simulink model "mars_rover_terrain"  (R2025a)
settings: Solver=daessc  StartTime=0.0  StopTime=130*10  FixedStep=1e-10  MaxStep=1e-1  RelTol=1e-3  AbsTol=1e-3  EnableMultiTasking=on
undefined symbols (not defined in the file): arm_q0, Control, eeConfig, L1, L2, L3, LS1, LS3, R1, R2, R3, Rover, rover_path, RS1, RS3, X, Y, Z
libraries: sm_lib x137, nesl_utility x109, fl_lib x85, sdl_lib x20, ee_lib x10, mars_rover_lib x8, simulink x4, slpidlib x3, batteryecm_lib x2, robotcorelib x1, robotalgslib x1
(part 3 of 10)

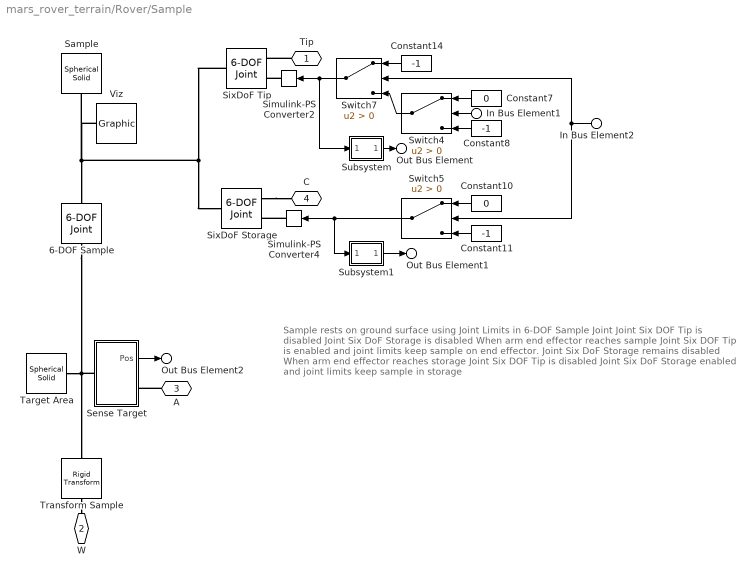
== system mars_rover_terrain/Rover/Sample ==
  note: Sample rests on ground surface using Joint Limits in 6-DOF Sample Joint
      | Joint Six DOF Tip is disabled
      | Joint Six DoF Storage is disabled
      |
      | When arm end effector reaches sample
      | Joint Six DOF Tip is enabled and joint limits keep sample on end effector.
      | Joint Six DoF Storage remains disabled
      |
      | When arm end effector reaches storage
      | Joint Six DOF Tip is disabled
      | Joint Six DoF Storage enabled and joint limits keep sample in storage
  In Bus Element1 : Inport  PortName=Ctrl  Element=Hold
  In Bus Element2 : Inport  PortName=Ctrl  Element=Stored
  6-DOF Sample : sm_lib/Joints/6-DOF Joint  JointMode=Normal  CompositeWrenchDir=FollowerOnBase  CompositeWrenchFrame=BaseFrame  SenseConstraintForce=off  SenseConstraintTorque=off  SenseTotalForce=off  SenseTotalTorque=off  PxPositionTargetSpecify=off  PxPositionTargetPriority=High  PxPositionTargetValue=0  PxPositionTargetValueUnits=m  PxVelocityTargetSpecify=off  PxVelocityTargetPriority=High  PxVelocityTargetValue=0  PxVelocityTargetValueUnits=m/s  PxEquilibriumPosition=0  PxEquilibriumPositionUnits=m  PxSpringStiffness=0  PxSpringStiffnessUnits=N/m  PxDampingCoefficient=0  PxDampingCoefficientUnits=N/(m/s)  PxLowerLimitSpecify=off  PxLowerLimitBound=-1  PxLowerLimitBoundUnits=m  PxLowerLimitStiffness=1e6  PxLowerLimitStiffnessUnits=N/m  PxLowerLimitDamping=1e3  PxLowerLimitDampingUnits=N/(m/s)  PxLowerLimitTransitionRegionWidth=1e-4  PxLowerLimitTransitionRegionWidthUnits=m  PxUpperLimitSpecify=off  PxUpperLimitBound=1  PxUpperLimitBoundUnits=m  PxUpperLimitStiffness=1e6  PxUpperLimitStiffnessUnits=N/m  PxUpperLimitDamping=1e3  PxUpperLimitDampingUnits=N/(m/s)  PxUpperLimitTransitionRegionWidth=1e-4  PxUpperLimitTransitionRegionWidthUnits=m  PxTorqueActuationMode=NoTorque  PxMotionActuationMode=ComputedMotion  PxSensePosition=off  PxSenseVelocity=off  PxSenseAcceleration=off  PxSenseTorqueForce=off  PxSenseLowerLimitTorqueForce=off  PxSenseUpperLimitTorqueForce=off  PyPositionTargetSpecify=off  PyPositionTargetPriority=High  PyPositionTargetValue=0  PyPositionTargetValueUnits=m  PyVelocityTargetSpecify=off  PyVelocityTargetPriority=High  PyVelocityTargetValue=0  PyVelocityTargetValueUnits=m/s  PyEquilibriumPosition=0  PyEquilibriumPositionUnits=m  PySpringStiffness=0  PySpringStiffnessUnits=N/m  PyDampingCoefficient=0  PyDampingCoefficientUnits=N/(m/s)  PyLowerLimitSpecify=off  PyLowerLimitBound=-1  PyLowerLimitBoundUnits=m  PyLowerLimitStiffness=1e6  PyLowerLimitStiffnessUnits=N/m  PyLowerLimitDamping=1e3  PyLowerLimitDampingUnits=N/(m/s)  PyLowerLimitTransitionRegionWidth=1e-4  PyLowerLimitTransitionRegionWidthUnits=m  PyUpperLimitSpecify=off  PyUpperLimitBound=1  PyUpperLimitBoundUnits=m  PyUpperLimitStiffness=1e6  PyUpperLimitStiffnessUnits=N/m  PyUpperLimitDamping=1e3  PyUpperLimitDampingUnits=N/(m/s)  PyUpperLimitTransitionRegionWidth=1e-4  PyUpperLimitTransitionRegionWidthUnits=m  PyTorqueActuationMode=NoTorque  PyMotionActuationMode=ComputedMotion  PySensePosition=off  PySenseVelocity=off  PySenseAcceleration=off  PySenseTorqueForce=off  PySenseLowerLimitTorqueForce=off  PySenseUpperLimitTorqueForce=off  PzPositionTargetSpecify=off  PzPositionTargetPriority=High  PzPositionTargetValue=0  PzPositionTargetValueUnits=m  PzVelocityTargetSpecify=off  PzVelocityTargetPriority=High  PzVelocityTargetValue=0  PzVelocityTargetValueUnits=m/s  PzEquilibriumPosition=0  PzEquilibriumPositionUnits=m  PzSpringStiffness=0  PzSpringStiffnessUnits=N/m  PzDampingCoefficient=0  PzDampingCoefficientUnits=N/(m/s)  PzLowerLimitSpecify=on  PzLowerLimitBound=0  PzLowerLimitBoundUnits=m  PzLowerLimitStiffness=1e6  PzLowerLimitStiffnessUnits=N/m  PzLowerLimitDamping=1e3  PzLowerLimitDampingUnits=N/(m/s)  PzLowerLimitTransitionRegionWidth=1e-4  PzLowerLimitTransitionRegionWidthUnits=m  PzUpperLimitSpecify=off  PzUpperLimitBound=1  PzUpperLimitBoundUnits=m  PzUpperLimitStiffness=1e6  PzUpperLimitStiffnessUnits=N/m  PzUpperLimitDamping=1e3  PzUpperLimitDampingUnits=N/(m/s)  PzUpperLimitTransitionRegionWidth=1e-4  PzUpperLimitTransitionRegionWidthUnits=m  PzTorqueActuationMode=NoTorque  PzMotionActuationMode=ComputedMotion  PzSensePosition=off  PzSenseVelocity=off  PzSenseAcceleration=off  PzSenseTorqueForce=off  PzSenseLowerLimitTorqueForce=off  PzSenseUpperLimitTorqueForce=off  SphPositionTargetSpecify=off  SphPositionTargetPriority=High  SphPositionTargetRotationMethod=None  SphPositionTargetFollAlignAxisA=+X  SphPositionTargetBaseAlignAxisA=+Y  SphPositionTargetFollAlignAxisB=+Y  SphPositionTargetBaseAlignAxisB=+Z  SphPositionTargetRotationStandardAxis=+Z  SphPositionTargetRotationAngle=0.0  SphPositionTargetRotationAngleUnits=deg  SphPositionTargetRotationArbitraryAxis=[0 0 1]  SphPositionTargetRotationSequenceAxes=FollowerAxes  SphPositionTargetRotationSequence=XYX  SphPositionTargetRotationSequenceAngles=[0 0 0]  SphPositionTargetRotationSequenceAnglesUnits=deg  SphPositionTargetRotationMatrix=[1 0 0; 0 1 0; 0 0 1]  SphPositionTargetQuaternion=[1 0 0 0]  SphVelocityTargetSpecify=off  SphVelocityTargetPriority=High  SphVelocityTargetValue=[0 0 0]  SphVelocityTargetValueUnits=deg/s  SphVelocityTargetInFollowerFrame=on  SphEqPosRotationMethod=None  SphEqPosFollAlignAxisA=+X  SphEqPosBaseAlignAxisA=+Y  SphEqPosFollAlignAxisB=+Y  SphEqPosBaseAlignAxisB=+Z  SphEqPosRotationStandardAxis=+Z  SphEqPosRotationAngle=0.0  SphEqPosRotationAngleUnits=deg  SphEqPosRotationArbitraryAxis=[0 0 1]  SphEqPosRotationSequenceAxes=FollowerAxes  SphEqPosRotationSequence=XYX  SphEqPosRotationSequenceAngles=[0 0 0]  SphEqPosRotationSequenceAnglesUnits=deg  SphEqPosRotationMatrix=[1 0 0; 0 1 0; 0 0 1]  SphEqPosQuaternion=[1 0 0 0]  SphSpringStiffness=0  SphSpringStiffnessUnits=N*m/deg  SphDampingCoefficient=0  SphDampingCoefficientUnits=N*m/(deg/s)  SphLowerLimitSpecify=off  SphLowerLimitBound=15  SphLowerLimitBoundUnits=deg  SphLowerLimitStiffness=1e4  SphLowerLimitStiffnessUnits=N*m/deg  SphLowerLimitDamping=10  SphLowerLimitDampingUnits=N*m/(deg/s)  SphLowerLimitTransitionRegionWidth=0.1  SphLowerLimitTransitionRegionWidthUnits=deg  SphUpperLimitSpecify=off  SphUpperLimitBound=45  SphUpperLimitBoundUnits=deg  SphUpperLimitStiffness=1e4  SphUpperLimitStiffnessUnits=N*m/deg  SphUpperLimitDamping=10  SphUpperLimitDampingUnits=N*m/(deg/s)  SphUpperLimitTransitionRegionWidth=0.1  SphUpperLimitTransitionRegionWidthUnits=deg  SphTorqueActuationMode=NoTorque  SphActuateTorqueX=off  SphActuateTorqueY=off  SphActuateTorqueZ=off  SphActuateTorque=off  SphActuationFrame=BaseFrame  SphSensePosition=off  SphSenseVelocityX=off  SphSenseVelocityY=off  SphSenseVelocityZ=off  SphSenseVelocity=off  SphSenseAccelerationX=off  SphSenseAccelerationY=off  SphSenseAccelerationZ=off  SphSenseAcceleration=off  SphSenseLowerLimitTorqueMag=off  SphSenseUpperLimitTorqueMag=off  SphSensingFrame=BaseFrame
  Constant10 : Constant  Value=0
  Constant11 : Constant  Value=-1
  Constant14 : Constant  Value=-1
  Constant7 : Constant  Value=0
  Constant8 : Constant  Value=-1
  Sample : sm_lib/Body Elements/Spherical Solid  SphereRadius=0.02  SphereRadiusUnits=m  ExportEntireGeometry=off  InertiaType=CalculateFromGeometry  BasedOnType=Density  Density=2582  DensityUnits=kg/m^3  Mass=0.001  MassUnits=kg  CenterOfMass=[0 0 0]  CenterOfMassUnits=m  MomentsOfInertia=[1 1 1]  MomentsOfInertiaUnits=kg*m^2  ProductsOfInertia=[0 0 0]  ProductsOfInertiaUnits=kg*m^2  GraphicType=FromGeometry  MarkerShape=Sphere  MarkerSize=10  GraphicVisPropType=AdvancedVisualProperties  GraphicDiffuseColor=[1 0 0]  GraphicOpacity=1.0  GraphicSpecularColor=[0.5 0.5 0.5 1.0]  GraphicAmbientColor=[0.15 0.15 0.15 1.0]  GraphicEmissiveColor=[0.0 0.0 0.0 1.0]  GraphicShininess=25  DoExposeReferenceFrame=on  SerializedFrames=<Frames/>
  Sense Target : Subsystem
  Simulink-PS Converter2 : nesl_utility/Simulink-PS Converter  PhysicalDomain=network_engine_domain  SubClassName=ps_input  LeftPortType=input  RightPortType=output  PseudoPeriodic=off  Frequencies=[]  NoiseDistribution=none  NoiseParameters=[]  Unit=1  AffineConversion=off  FilteringAndDerivatives=provide  SimscapeFilterOrder=1  InputFilterTimeConstant=0.001  UdotUserProvided=0
  Simulink-PS Converter4 : nesl_utility/Simulink-PS Converter  PhysicalDomain=network_engine_domain  SubClassName=ps_input  LeftPortType=input  RightPortType=output  PseudoPeriodic=off  Frequencies=[]  NoiseDistribution=none  NoiseParameters=[]  Unit=1  AffineConversion=off  FilteringAndDerivatives=provide  SimscapeFilterOrder=1  InputFilterTimeConstant=0.001  UdotUserProvided=0
  SixDoF Storage : sm_lib/Joints/6-DOF Joint  JointMode=ProvidedByInput  CompositeWrenchDir=FollowerOnBase  CompositeWrenchFrame=BaseFrame  SenseConstraintForce=off  SenseConstraintTorque=off  SenseTotalForce=off  SenseTotalTorque=off  PxPositionTargetSpecify=off  PxPositionTargetPriority=High  PxPositionTargetValue=0  PxPositionTargetValueUnits=m  PxVelocityTargetSpecify=off  PxVelocityTargetPriority=High  PxVelocityTargetValue=0  PxVelocityTargetValueUnits=m/s  PxEquilibriumPosition=0  PxEquilibriumPositionUnits=m  PxSpringStiffness=0  PxSpringStiffnessUnits=N/m  PxDampingCoefficient=0.1  PxDampingCoefficientUnits=N/(m/s)  PxLowerLimitSpecify=on  PxLowerLimitBound=-0.01  PxLowerLimitBoundUnits=m  PxLowerLimitStiffness=1e4  PxLowerLimitStiffnessUnits=N/m  PxLowerLimitDamping=1e2  PxLowerLimitDampingUnits=N/(m/s)  PxLowerLimitTransitionRegionWidth=1e-3  PxLowerLimitTransitionRegionWidthUnits=m  PxUpperLimitSpecify=on  PxUpperLimitBound=0.01  PxUpperLimitBoundUnits=m  PxUpperLimitStiffness=1e4  PxUpperLimitStiffnessUnits=N/m  PxUpperLimitDamping=1e2  PxUpperLimitDampingUnits=N/(m/s)  PxUpperLimitTransitionRegionWidth=1e-3  PxUpperLimitTransitionRegionWidthUnits=m  PxTorqueActuationMode=NoTorque  PxMotionActuationMode=ComputedMotion  PxSensePosition=off  PxSenseVelocity=off  PxSenseAcceleration=off  PxSenseTorqueForce=off  PxSenseLowerLimitTorqueForce=off  PxSenseUpperLimitTorqueForce=off  PyPositionTargetSpecify=off  PyPositionTargetPriority=High  PyPositionTargetValue=0  PyPositionTargetValueUnits=m  PyVelocityTargetSpecify=off  PyVelocityTargetPriority=High  PyVelocityTargetValue=0  PyVelocityTargetValueUnits=m/s  PyEquilibriumPosition=0  PyEquilibriumPositionUnits=m  PySpringStiffness=0  PySpringStiffnessUnits=N/m  PyDampingCoefficient=0.1  PyDampingCoefficientUnits=N/(m/s)  PyLowerLimitSpecify=on  PyLowerLimitBound=-0.01  PyLowerLimitBoundUnits=m  PyLowerLimitStiffness=1e4  PyLowerLimitStiffnessUnits=N/m  PyLowerLimitDamping=1e3  PyLowerLimitDampingUnits=N/(m/s)  PyLowerLimitTransitionRegionWidth=1e-3  PyLowerLimitTransitionRegionWidthUnits=m  PyUpperLimitSpecify=on  PyUpperLimitBound=0.01  PyUpperLimitBoundUnits=m  PyUpperLimitStiffness=1e4  PyUpperLimitStiffnessUnits=N/m  PyUpperLimitDamping=1e3  PyUpperLimitDampingUnits=N/(m/s)  PyUpperLimitTransitionRegionWidth=1e-3  PyUpperLimitTransitionRegionWidthUnits=m  PyTorqueActuationMode=NoTorque  PyMotionActuationMode=ComputedMotion  PySensePosition=off  PySenseVelocity=off  PySenseAcceleration=off  PySenseTorqueForce=off  PySenseLowerLimitTorqueForce=off  PySenseUpperLimitTorqueForce=off  PzPositionTargetSpecify=off  PzPositionTargetPriority=High  PzPositionTargetValue=0  PzPositionTargetValueUnits=m  PzVelocityTargetSpecify=off  PzVelocityTargetPriority=High  PzVelocityTargetValue=0  PzVelocityTargetValueUnits=m/s  PzEquilibriumPosition=0  PzEquilibriumPositionUnits=m  PzSpringStiffness=0  PzSpringStiffnessUnits=N/m  PzDampingCoefficient=0.1  PzDampingCoefficientUnits=N/(m/s)  PzLowerLimitSpecify=on  PzLowerLimitBound=-0.02  PzLowerLimitBoundUnits=m  PzLowerLimitStiffness=1e4  PzLowerLimitStiffnessUnits=N/m  PzLowerLimitDamping=1e3  PzLowerLimitDampingUnits=N/(m/s)  PzLowerLimitTransitionRegionWidth=1e-3  PzLowerLimitTransitionRegionWidthUnits=m  PzUpperLimitSpecify=on  PzUpperLimitBound=0.02  PzUpperLimitBoundUnits=m  PzUpperLimitStiffness=1e4  PzUpperLimitStiffnessUnits=N/m  PzUpperLimitDamping=1e3  PzUpperLimitDampingUnits=N/(m/s)  PzUpperLimitTransitionRegionWidth=1e-3  PzUpperLimitTransitionRegionWidthUnits=m  PzTorqueActuationMode=NoTorque  PzMotionActuationMode=ComputedMotion  PzSensePosition=off  PzSenseVelocity=off  PzSenseAcceleration=off  PzSenseTorqueForce=off  PzSenseLowerLimitTorqueForce=off  PzSenseUpperLimitTorqueForce=off  SphPositionTargetSpecify=off  SphPositionTargetPriority=High  SphPositionTargetRotationMethod=None  SphPositionTargetFollAlignAxisA=+X  SphPositionTargetBaseAlignAxisA=+Y  SphPositionTargetFollAlignAxisB=+Y  SphPositionTargetBaseAlignAxisB=+Z  SphPositionTargetRotationStandardAxis=+Z  SphPositionTargetRotationAngle=0.0  SphPositionTargetRotationAngleUnits=deg  SphPositionTargetRotationArbitraryAxis=[0 0 1]  SphPositionTargetRotationSequenceAxes=FollowerAxes  SphPositionTargetRotationSequence=XYX  SphPositionTargetRotationSequenceAngles=[0 0 0]  SphPositionTargetRotationSequenceAnglesUnits=deg  SphPositionTargetRotationMatrix=[1 0 0; 0 1 0; 0 0 1]  SphPositionTargetQuaternion=[1 0 0 0]  SphVelocityTargetSpecify=off  SphVelocityTargetPriority=High  SphVelocityTargetValue=[0 0 0]  SphVelocityTargetValueUnits=deg/s  SphVelocityTargetInFollowerFrame=on  SphEqPosRotationMethod=None  SphEqPosFollAlignAxisA=+X  SphEqPosBaseAlignAxisA=+Y  SphEqPosFollAlignAxisB=+Y  SphEqPosBaseAlignAxisB=+Z  SphEqPosRotationStandardAxis=+Z  SphEqPosRotationAngle=0.0  SphEqPosRotationAngleUnits=deg  SphEqPosRotationArbitraryAxis=[0 0 1]  SphEqPosRotationSequenceAxes=FollowerAxes  SphEqPosRotationSequence=XYX  SphEqPosRotationSequenceAngles=[0 0 0]  SphEqPosRotationSequenceAnglesUnits=deg  SphEqPosRotationMatrix=[1 0 0; 0 1 0; 0 0 1]  SphEqPosQuaternion=[1 0 0 0]  SphSpringStiffness=0  SphSpringStiffnessUnits=N*m/deg  SphDampingCoefficient=0.1  SphDampingCoefficientUnits=N*m/(deg/s)  SphLowerLimitSpecify=off  SphLowerLimitBound=15  SphLowerLimitBoundUnits=deg  SphLowerLimitStiffness=1e4  SphLowerLimitStiffnessUnits=N*m/deg  SphLowerLimitDamping=10  SphLowerLimitDampingUnits=N*m/(deg/s)  SphLowerLimitTransitionRegionWidth=0.1  SphLowerLimitTransitionRegionWidthUnits=deg  SphUpperLimitSpecify=off  SphUpperLimitBound=45  SphUpperLimitBoundUnits=deg  SphUpperLimitStiffness=1e4  SphUpperLimitStiffnessUnits=N*m/deg  SphUpperLimitDamping=10  SphUpperLimitDampingUnits=N*m/(deg/s)  SphUpperLimitTransitionRegionWidth=0.1  SphUpperLimitTransitionRegionWidthUnits=deg  SphTorqueActuationMode=NoTorque  SphActuateTorqueX=off  SphActuateTorqueY=off  SphActuateTorqueZ=off  SphActuateTorque=off  SphActuationFrame=BaseFrame  SphSensePosition=off  SphSenseVelocityX=off  SphSenseVelocityY=off  SphSenseVelocityZ=off  SphSenseVelocity=off  SphSenseAccelerationX=off  SphSenseAccelerationY=off  SphSenseAccelerationZ=off  SphSenseAcceleration=off  SphSenseLowerLimitTorqueMag=off  SphSenseUpperLimitTorqueMag=off  SphSensingFrame=BaseFrame
  SixDoF Tip : sm_lib/Joints/6-DOF Joint  JointMode=ProvidedByInput  CompositeWrenchDir=FollowerOnBase  CompositeWrenchFrame=BaseFrame  SenseConstraintForce=off  SenseConstraintTorque=off  SenseTotalForce=off  SenseTotalTorque=off  PxPositionTargetSpecify=off  PxPositionTargetPriority=High  PxPositionTargetValue=0  PxPositionTargetValueUnits=m  PxVelocityTargetSpecify=off  PxVelocityTargetPriority=High  PxVelocityTargetValue=0  PxVelocityTargetValueUnits=m/s  PxEquilibriumPosition=0  PxEquilibriumPositionUnits=m  PxSpringStiffness=0  PxSpringStiffnessUnits=N/m  PxDampingCoefficient=0.1  PxDampingCoefficientUnits=N/(m/s)  PxLowerLimitSpecify=on  PxLowerLimitBound=-Rover.Arm.Tip.lim.bound  PxLowerLimitBoundUnits=m  PxLowerLimitStiffness=Rover.Arm.Tip.lim.k  PxLowerLimitStiffnessUnits=N/m  PxLowerLimitDamping=Rover.Arm.Tip.lim.d  PxLowerLimitDampingUnits=N/(m/s)  PxLowerLimitTransitionRegionWidth=Rover.Arm.Tip.lim.w  PxLowerLimitTransitionRegionWidthUnits=m  PxUpperLimitSpecify=on  PxUpperLimitBound=Rover.Arm.Tip.lim.bound  PxUpperLimitBoundUnits=m  PxUpperLimitStiffness=Rover.Arm.Tip.lim.k  PxUpperLimitStiffnessUnits=N/m  PxUpperLimitDamping=Rover.Arm.Tip.lim.d  PxUpperLimitDampingUnits=N/(m/s)  PxUpperLimitTransitionRegionWidth=Rover.Arm.Tip.lim.w  PxUpperLimitTransitionRegionWidthUnits=m  PxTorqueActuationMode=NoTorque  PxMotionActuationMode=ComputedMotion  PxSensePosition=off  PxSenseVelocity=off  PxSenseAcceleration=off  PxSenseTorqueForce=off  PxSenseLowerLimitTorqueForce=off  PxSenseUpperLimitTorqueForce=off  PyPositionTargetSpecify=off  PyPositionTargetPriority=High  PyPositionTargetValue=0  PyPositionTargetValueUnits=m  PyVelocityTargetSpecify=off  PyVelocityTargetPriority=High  PyVelocityTargetValue=0  PyVelocityTargetValueUnits=m/s  PyEquilibriumPosition=0  PyEquilibriumPositionUnits=m  PySpringStiffness=0  PySpringStiffnessUnits=N/m  PyDampingCoefficient=0.1  PyDampingCoefficientUnits=N/(m/s)  PyLowerLimitSpecify=on  PyLowerLimitBound=-Rover.Arm.Tip.lim.bound  PyLowerLimitBoundUnits=m  PyLowerLimitStiffness=Rover.Arm.Tip.lim.k  PyLowerLimitStiffnessUnits=N/m  PyLowerLimitDamping=Rover.Arm.Tip.lim.d  PyLowerLimitDampingUnits=N/(m/s)  PyLowerLimitTransitionRegionWidth=Rover.Arm.Tip.lim.w  PyLowerLimitTransitionRegionWidthUnits=m  PyUpperLimitSpecify=on  PyUpperLimitBound=Rover.Arm.Tip.lim.bound  PyUpperLimitBoundUnits=m  PyUpperLimitStiffness=Rover.Arm.Tip.lim.k  PyUpperLimitStiffnessUnits=N/m  PyUpperLimitDamping=Rover.Arm.Tip.lim.d  PyUpperLimitDampingUnits=N/(m/s)  PyUpperLimitTransitionRegionWidth=Rover.Arm.Tip.lim.w  PyUpperLimitTransitionRegionWidthUnits=m  PyTorqueActuationMode=NoTorque  PyMotionActuationMode=ComputedMotion  PySensePosition=off  PySenseVelocity=off  PySenseAcceleration=off  PySenseTorqueForce=off  PySenseLowerLimitTorqueForce=off  PySenseUpperLimitTorqueForce=off  PzPositionTargetSpecify=off  PzPositionTargetPriority=High  PzPositionTargetValue=0  PzPositionTargetValueUnits=m  PzVelocityTargetSpecify=off  PzVelocityTargetPriority=High  PzVelocityTargetValue=0  PzVelocityTargetValueUnits=m/s  PzEquilibriumPosition=0  PzEquilibriumPositionUnits=m  PzSpringStiffness=0  PzSpringStiffnessUnits=N/m  PzDampingCoefficient=0.1  PzDampingCoefficientUnits=N/(m/s)  PzLowerLimitSpecify=on  PzLowerLimitBound=-Rover.Arm.Tip.lim.bound  PzLowerLimitBoundUnits=m  PzLowerLimitStiffness=Rover.Arm.Tip.lim.k  PzLowerLimitStiffnessUnits=N/m  PzLowerLimitDamping=Rover.Arm.Tip.lim.d  PzLowerLimitDampingUnits=N/(m/s)  PzLowerLimitTransitionRegionWidth=Rover.Arm.Tip.lim.w  PzLowerLimitTransitionRegionWidthUnits=m  PzUpperLimitSpecify=on  PzUpperLimitBound=Rover.Arm.Tip.lim.bound  PzUpperLimitBoundUnits=m  PzUpperLimitStiffness=Rover.Arm.Tip.lim.k  PzUpperLimitStiffnessUnits=N/m  PzUpperLimitDamping=Rover.Arm.Tip.lim.d  PzUpperLimitDampingUnits=N/(m/s)  PzUpperLimitTransitionRegionWidth=Rover.Arm.Tip.lim.w  PzUpperLimitTransitionRegionWidthUnits=m  PzTorqueActuationMode=NoTorque  PzMotionActuationMode=ComputedMotion  PzSensePosition=off  PzSenseVelocity=off  PzSenseAcceleration=off  PzSenseTorqueForce=off  PzSenseLowerLimitTorqueForce=off  PzSenseUpperLimitTorqueForce=off  SphPositionTargetSpecify=off  SphPositionTargetPriority=High  SphPositionTargetRotationMethod=None  SphPositionTargetFollAlignAxisA=+X  SphPositionTargetBaseAlignAxisA=+Y  SphPositionTargetFollAlignAxisB=+Y  SphPositionTargetBaseAlignAxisB=+Z  SphPositionTargetRotationStandardAxis=+Z  SphPositionTargetRotationAngle=0.0  SphPositionTargetRotationAngleUnits=deg  SphPositionTargetRotationArbitraryAxis=[0 0 1]  SphPositionTargetRotationSequenceAxes=FollowerAxes  SphPositionTargetRotationSequence=XYX  SphPositionTargetRotationSequenceAngles=[0 0 0]  SphPositionTargetRotationSequenceAnglesUnits=deg  SphPositionTargetRotationMatrix=[1 0 0; 0 1 0; 0 0 1]  SphPositionTargetQuaternion=[1 0 0 0]  SphVelocityTargetSpecify=off  SphVelocityTargetPriority=High  SphVelocityTargetValue=[0 0 0]  SphVelocityTargetValueUnits=deg/s  SphVelocityTargetInFollowerFrame=on  SphEqPosRotationMethod=None  SphEqPosFollAlignAxisA=+X  SphEqPosBaseAlignAxisA=+Y  SphEqPosFollAlignAxisB=+Y  SphEqPosBaseAlignAxisB=+Z  SphEqPosRotationStandardAxis=+Z  SphEqPosRotationAngle=0.0  SphEqPosRotationAngleUnits=deg  SphEqPosRotationArbitraryAxis=[0 0 1]  SphEqPosRotationSequenceAxes=FollowerAxes  SphEqPosRotationSequence=XYX  SphEqPosRotationSequenceAngles=[0 0 0]  SphEqPosRotationSequenceAnglesUnits=deg  SphEqPosRotationMatrix=[1 0 0; 0 1 0; 0 0 1]  SphEqPosQuaternion=[1 0 0 0]  SphSpringStiffness=0  SphSpringStiffnessUnits=N*m/deg  SphDampingCoefficient=0  SphDampingCoefficientUnits=N*m/(deg/s)  SphLowerLimitSpecify=off  SphLowerLimitBound=15  SphLowerLimitBoundUnits=deg  SphLowerLimitStiffness=1e4  SphLowerLimitStiffnessUnits=N*m/deg  SphLowerLimitDamping=10  SphLowerLimitDampingUnits=N*m/(deg/s)  SphLowerLimitTransitionRegionWidth=0.1  SphLowerLimitTransitionRegionWidthUnits=deg  SphUpperLimitSpecify=off  SphUpperLimitBound=45  SphUpperLimitBoundUnits=deg  SphUpperLimitStiffness=1e4  SphUpperLimitStiffnessUnits=N*m/deg  SphUpperLimitDamping=10  SphUpperLimitDampingUnits=N*m/(deg/s)  SphUpperLimitTransitionRegionWidth=0.1  SphUpperLimitTransitionRegionWidthUnits=deg  SphTorqueActuationMode=NoTorque  SphActuateTorqueX=off  SphActuateTorqueY=off  SphActuateTorqueZ=off  SphActuateTorque=off  SphActuationFrame=BaseFrame  SphSensePosition=off  SphSenseVelocityX=off  SphSenseVelocityY=off  SphSenseVelocityZ=off  SphSenseVelocity=off  SphSenseAccelerationX=off  SphSenseAccelerationY=off  SphSenseAccelerationZ=off  SphSenseAcceleration=off  SphSenseLowerLimitTorqueMag=off  SphSenseUpperLimitTorqueMag=off  SphSensingFrame=BaseFrame
  Subsystem : Subsystem
  Subsystem1 : Subsystem
  Switch4 : Switch  Criteria=u2 > Threshold  SaturateOnIntegerOverflow=off  InputSameDT=off
  Switch5 : Switch  Criteria=u2 > Threshold  SaturateOnIntegerOverflow=off  InputSameDT=off
  Switch7 : Switch  Criteria=u2 > Threshold  SaturateOnIntegerOverflow=off  InputSameDT=off
  Target Area : sm_lib/Body Elements/Spherical Solid  SphereRadius=0.35  SphereRadiusUnits=m  ExportEntireGeometry=off  InertiaType=CalculateFromGeometry  BasedOnType=Density  Density=1000  DensityUnits=kg/m^3  Mass=1  MassUnits=kg  CenterOfMass=[0 0 0]  CenterOfMassUnits=m  MomentsOfInertia=[1 1 1]  MomentsOfInertiaUnits=kg*m^2  ProductsOfInertia=[0 0 0]  ProductsOfInertiaUnits=kg*m^2  GraphicType=FromGeometry  MarkerShape=Sphere  MarkerSize=10  GraphicVisPropType=SimpleVisualProperties  GraphicDiffuseColor=[0.4 1.0 0.2]  GraphicOpacity=0.3  GraphicSpecularColor=[0.5 0.5 0.5 1.0]  GraphicAmbientColor=[0.15 0.15 0.15 1.0]  GraphicEmissiveColor=[0.0 0.0 0.0 1.0]  GraphicShininess=75  DoExposeReferenceFrame=on  SerializedFrames=<Frames/>
  Transform Sample : sm_lib/Frames and Transforms/Rigid Transform  RotationMethod=None  FollAlignAxisA=+X  BaseAlignAxisA=+Y  FollAlignAxisB=+Y  BaseAlignAxisB=+Z  RotationStandardAxis=+Z  RotationAngle=0.0  RotationAngleUnits=deg  RotationArbitraryAxis=[0 0 1]  RotationSequenceAxes=FollowerAxes  RotationSequence=XYX  RotationSequenceAngles=[0 0 0]  RotationSequenceAnglesUnits=deg  RotationMatrix=[1 0 0; 0 1 0; 0 0 1]  Quaternion=[1 0 0 0]  TranslationMethod=Cartesian  TranslationCartesianOffset=sample_position  TranslationCartesianOffsetUnits=m  TranslationStandardAxis=+Z  TranslationStandardOffset=0  TranslationStandardOffsetUnits=m  TranslationROffset=0  TranslationROffsetUnits=m  TranslationThetaOffset=0  TranslationThetaOffsetUnits=deg  TranslationZOffset=0  TranslationZOffsetUnits=m
  Viz : sm_lib/Body Elements/Graphic  GraphicType=Marker  MarkerShape=Frame  MarkerSize=5  GraphicVisPropType=SimpleVisualProperties  GraphicDiffuseColor=[1 0 0]  GraphicOpacity=1.0  GraphicSpecularColor=[0.5 0.5 0.5 1.0]  GraphicAmbientColor=[0.15 0.15 0.15 1.0]  GraphicEmissiveColor=[0.0 0.0 0.0 1.0]  GraphicShininess=75
  Tip : PMIOPort  Side=Right
  W : PMIOPort  Port=2  Side=Left
  A : PMIOPort  Port=3  Side=Right
  C : PMIOPort  Port=4  Side=Right
  Out Bus Element : Outport  PortName=m  Element=SampleTip
  Out Bus Element1 : Outport  PortName=m  Element=SampleStorage
  Out Bus Element2 : Outport  PortName=m  Element=TargetChassis
  wires:
  Constant7/1 -> Switch4/1
  Constant8/1 -> Switch4/3
  In Bus Element2/1 -> Switch5/2, Switch7/2
  Constant11/1 -> Switch5/3
  Constant10/1 -> Switch5/1
  Switch4/1 -> Switch7/3
  Switch5/1 -> Subsystem1/1(In1), Simulink-PS Converter4/1
  In Bus Element1/1 -> Switch4/2
  Constant14/1 -> Switch7/1
  Switch7/1 -> Subsystem/1(In1), Simulink-PS Converter2/1
  Subsystem/1(Out1) -> Out Bus Element/1
  Sense Target/1(Pos) -> Out Bus Element2/1
  Subsystem1/1(m) -> Out Bus Element1/1
  connections:
  SixDoF Tip/RConn1 -- Viz/RConn1 -- Sample/RConn1 -- 6-DOF Sample/RConn1 -- SixDoF Storage/RConn1
  Simulink-PS Converter4/RConn1 -- SixDoF Storage/LConn2
  SixDoF Storage/LConn1 -- C/RConn1
  6-DOF Sample/LConn1 -- Target Area/RConn1 -- Transform Sample/RConn1 -- Sense Target/LConn1
  Simulink-PS Converter2/RConn1 -- SixDoF Tip/LConn2
  Tip/RConn1 -- SixDoF Tip/LConn1
  A/RConn1 -- Sense Target/RConn1
  Transform Sample/LConn1 -- W/RConn1

== system mars_rover_terrain/Rover/Terrain ==
  note: Uncomment for additional terrain visualization options.
  Contact : Subsystem  mask{contact_k=Rover.Wheel_Surface.Contact.k, contact_d=Rover.Wheel_Surface.Contact.d, contact_tw=Rover.Wheel_Surface.Contact.trans_depth, friction_mus=Rover.Wheel_Surface.Friction.mu_static, friction_mud=Rover.Wheel_Surface.Friction.mu_dynamic, friction_vcrit=Rover.Wheel_Surface.Friction.vel_crit}
      mask prompts: contact_k "Stiffness (N/m)"; contact_d "Damping (N/(m/s))"; contact_tw "Transition Region Width (m)"; friction_mus "Coefficient of Static Friction"; friction_mud "Coefficient of Dynamic Friction"; friction_vcrit "Critical Velocity (m/s)"
      mask DialogControl cont_contact Prompt: Contact Parameters
      mask DialogControl cont_friction Prompt: Contact Friction
  Terrain Geometry : sm_lib/Body Elements/File Solid  Commented=on  ExtGeomFileName=mars_terrain.stl  UnitType=Custom  ExtGeomFileUnits=m  StepReaderType=HEX  ExportConvexHullGeometry=off  InertiaType=CalculateFromGeometry  BasedOnType=Mass  Density=1000  DensityUnits=kg/m^3  Mass=1  MassUnits=kg  CenterOfMass=[0 0 0]  CenterOfMassUnits=m  MomentsOfInertia=[1 1 1]  MomentsOfInertiaUnits=kg*m^2  ProductsOfInertia=[0 0 0]  ProductsOfInertiaUnits=kg*m^2  GraphicType=FromGeometry  MarkerShape=Sphere  MarkerSize=10  GraphicVisPropType=SimpleVisualProperties  GraphicDiffuseColor=[1.0 0.6 0.6]  GraphicOpacity=1.0  GraphicSpecularColor=[0.5 0.5 0.5 1.0]  GraphicAmbientColor=[0.15 0.15 0.15 1.0]  GraphicEmissiveColor=[0.0 0.0 0.0 1.0]  GraphicShininess=75  DoExposeReferenceFrame=on  SerializedFrames=<Frames/>
  Terrain Point Cloud : sm_lib/Curves and Surfaces/Point Cloud  Commented=on  CoordinatesMatrix=mars_terrain_grid.ptcloud  CoordinatesMatrixUnits=m  GraphicType=MarkerCloud  GraphicSphereRadius=0.03  GraphicSphereRadiusUnits=m  GraphicVisPropType=SimpleVisualProperties  GraphicDiffuseColor=[0 1 0]  GraphicOpacity=1.0  GraphicSpecularColor=[0.5 0.5 0.5 1.0]  GraphicAmbientColor=[0.15 0.15 0.15 1.0]  GraphicEmissiveColor=[0.0 0.0 0.0 1.0]  GraphicShininess=75
  Terrain Grid Surface : sm_lib/Curves and Surfaces/Grid Surface  XGridVector=mars_terrain_grid.xg  XGridVectorUnits=m  YGridVector=mars_terrain_grid.yg  YGridVectorUnits=m  ZHeights=mars_terrain_grid.z_heights  ZHeightsUnits=m  GraphicType=FromGeometry  GraphicVisPropType=SimpleVisualProperties  GraphicDiffuseColor=[187 109 63]/255*1.3  GraphicOpacity=1  GraphicSpecularColor=[0.5 0.5 0.5 1.0]  GraphicAmbientColor=[0.15 0.15 0.15 1.0]  GraphicEmissiveColor=[0.0 0.0 0.0 1.0]  GraphicShininess=75
  W : PMIOPort  Side=Right
  G : PMIOPort  Port=2  Side=Right
  connections:
  W/RConn1 -- Terrain Point Cloud/LConn1 -- Terrain Geometry/RConn1 -- Terrain Grid Surface/LConn1
  Contact/RConn1 -- G/RConn1
  Contact/RConn2 -- Terrain Grid Surface/RConn1

== system mars_rover_terrain/Control/Arm Control/ Trajectory Planner ==
  RoverAtGoal : Inport
  In Bus Element1 : Inport  Port=2  PortName=Sensing  Element=SampleTip
  In Bus Element2 : Inport  Port=2  PortName=Sensing  Element=SampleStorage
  In Bus Element3 : Inport  Port=2  PortName=Sensing  Element=TargetChassis
  Arm Angles : Inport  Port=3
  Check Drift : Subsystem
  Delay Arm Movement : Delay
  Delay Sample Check : Delay
  Planner Subsystem : Subsystem
  SampleDropOffCmdLogic : Subsystem
  SampleLoc wrt arm base : Subsystem
  SamplePickUpCmdLogic : Subsystem
  Scope : Scope  NumInputPorts=2
      settings: ActiveDisplayYMinimum=-0.125  ActiveDisplayYMaximum=1.125
  Switch : Switch  Criteria=u2 > Threshold  SaturateOnIntegerOverflow=off  InputSameDT=off
  hold1 : Subsystem
  hold2 : Subsystem
  q0 Arm : Constant  Value=arm_q0
  Hold : Outport
  Stored : Outport  Port=2
  Location : Outport  Port=3
  Mode : Outport  Port=4
  Cmd Angles : Outport  Port=5
  wires:
  Switch/1 -> Cmd Angles/1
  q0 Arm/1 -> Switch/3
  In Bus Element3/1 -> SampleLoc wrt arm base/2(SampleLoc), Check Drift/1(Sensor)
  Delay Arm Movement/1 -> Switch/2
  Arm Angles/1 -> Planner Subsystem/1(qJoints)
  SampleLoc wrt arm base/1(SamplePos) -> Check Drift/2(IK Target), Location/1, Planner Subsystem/2(SamplePosition)
  Planner Subsystem/2(CmdHold) -> SamplePickUpCmdLogic/1(u)
  Planner Subsystem/3(CmdStored) -> SampleDropOffCmdLogic/1(u)
  In Bus Element1/1 -> hold2/1(Enable)
  In Bus Element2/1 -> hold1/1(Enable)
  Planner Subsystem/1(qCmd) -> Switch/1
  hold2/1(plan) -> Planner Subsystem/3(Hold)
  hold1/1(plan) -> Planner Subsystem/4(Stored)
  SampleDropOffCmdLogic/1(y) -> Scope/2, Stored/1
  SamplePickUpCmdLogic/1(y) -> Scope/1, Hold/1
  Delay Sample Check/1 -> SampleLoc wrt arm base/1(Enable), Delay Arm Movement/1, Planner Subsystem/Enable
  RoverAtGoal/1 -> Delay Sample Check/1
  Planner Subsystem/4(Rover Mode) -> Mode/1

== system mars_rover_terrain/Control/Arm Control/Bus to Vec q ==
  B : Inport
  Bus Selector : BusSelector  OutputSignals=q.q1,q.q2,q.q3,q.q4,q.q5,q.q6
  Mux : Mux  Inputs=6
  V : Outport
  wires:
  Bus Selector/6 -> Mux/6  "<q6>"
  Bus Selector/4 -> Mux/4  "<q4>"
  Mux/1 -> V/1
  B/1 -> Bus Selector/1
  Bus Selector/1 -> Mux/1  "<q1>"
  Bus Selector/3 -> Mux/3  "<q3>"
  Bus Selector/2 -> Mux/2  "<q2>"
  Bus Selector/5 -> Mux/5  "<q5>"

== system mars_rover_terrain/Control/Arm Control/Vec to Bus q ==
  V : Inport
  Bus Creator : BusCreator  Inputs=6
  Demux : Demux  Outputs=6
  B : Outport
  wires:
  Demux/3 -> Bus Creator/3  "q3"
  Bus Creator/1 -> B/1
  V/1 -> Demux/1
  Demux/4 -> Bus Creator/4  "q4"
  Demux/1 -> Bus Creator/1  "q1"
  Demux/6 -> Bus Creator/6  "q6"
  Demux/2 -> Bus Creator/2  "q2"
  Demux/5 -> Bus Creator/5  "q5"

== system mars_rover_terrain/Control/Arm Control/Vec to Bus trq ==
  V : Inport
  Bus Creator : BusCreator  Inputs=6
  Demux : Demux  Outputs=6
  B : Outport
  wires:
  Demux/5 -> Bus Creator/5  "t5"
  Demux/2 -> Bus Creator/2  "t2"
  Demux/6 -> Bus Creator/6  "t6"
  Demux/1 -> Bus Creator/1  "t1"
  Demux/4 -> Bus Creator/4  "t4"
  V/1 -> Demux/1
  Bus Creator/1 -> B/1
  Demux/3 -> Bus Creator/3  "t3"

== system mars_rover_terrain/Control/Chassis Control/Ackerman Steer Angle ==
  note: ROC: Radius of Curvature
      | A3: Axle 3
      | L3: Rear Left Wheel
      | R3: Rear Right Wheel
  AtGoal : Inport
  Delta : Inport  Port=2
  Ackerman Steering Angle Formulation : MATLAB Function  TreatAsAtomicUnit=on
  Clock1 : Clock
  Constant : Constant  Value=Rover.Chassis.Length/2
  Constant3 : Constant  Value=0
  Constant4 : Constant  Value=Rover.Chassis.Width
  Gain3 : Gain  Gain=-1
  Gain4 : Gain  Gain=-1
  Hold Steer at Goal : Subsystem  TreatAsAtomicUnit=on
  Mux : Mux
  NOT : Logic  Operator=NOT  IconShape=distinctive  AllPortsSameDT=off  OutDataTypeStr=boolean
  Saturation{1..4} (4 alike) : Saturate  UpperLimit=60  LowerLimit=-60
  Scope : Scope  NumInputPorts=3
      settings: ActiveDisplayYMinimum=-35.60933  ActiveDisplayYMaximum=51.25577  DataLoggingVariableName=ScopeData2
  Switch2 : Switch  Criteria=u2 > Threshold  Threshold=1  SaturateOnIntegerOverflow=off  InputSameDT=off
  AckSteerAngs : Outport
  A3 ROC : Outport  Port=2
  L3ROC : Outport  Port=3
  R3ROC : Outport  Port=4
  wires:
  Delta/1 -> Switch2/1
  Ackerman Steering Angle Formulation/2(qSteerR3) -> Scope/3, Saturation3/1, Gain4/1
  Ackerman Steering Angle Formulation/5(R_R) -> R3ROC/1
  Saturation4/1 -> Mux/4  "R1"
  Saturation1/1 -> Mux/2  "L1"
  Hold Steer at Goal/1(d_h) -> Scope/1, Ackerman Steering Angle Formulation/1(delta)
  Ackerman Steering Angle Formulation/1(qSteerL3) -> Scope/2, Saturation2/1, Gain3/1
  Constant/1 -> Ackerman Steering Angle Formulation/2(L)
  Saturation3/1 -> Mux/3  "R3"
  Mux/1 -> AckSteerAngs/1
  Clock1/1 -> Switch2/2
  Switch2/1 -> Hold Steer at Goal/1(d)
  Gain4/1 -> Saturation4/1
  Saturation2/1 -> Mux/1  "L3"
  Constant4/1 -> Ackerman Steering Angle Formulation/3(d)
  Gain3/1 -> Saturation1/1
  Ackerman Steering Angle Formulation/4(L_R) -> L3ROC/1
  Ackerman Steering Angle Formulation/3(R) -> A3 ROC/1
  Constant3/1 -> Switch2/3
  AtGoal/1 -> NOT/1
  NOT/1 -> Hold Steer at Goal/Enable

== system mars_rover_terrain/Control/Chassis Control/Steering Controller ==
  Meas : Inport
  qSteerWhl : Inport  Port=2
  RoverAtGoal : Inport  Port=3
  Add : Sum  Inputs=+-
  Bus to Vec : Subsystem
  Check Difference : Subsystem
  Constant : Constant  Value=[Kp Ki]
  Constant1 : Constant  Value=[10 1 ]
  Constant2 : Constant  Value=Kd
  Constant3 : Constant  Value=N
  Demux : Demux  Outputs=2
  Demux1 : Demux
  Filter qMeas : Subsystem  mask(First-order lag supporting vector signals){b=[1 1 1 1]*Ts_Measq, x_initial=[0 0 0 0]}
      mask prompts: b "Filter time constant"; x_initial "Initial output"
      mask help: Models a lag of the form 1/(b*s+1) where s is the Laplace operator.
  Filter qTarget : Subsystem  mask(First-order lag supporting vector signals){b=[1 1 1 1]*Ts_Targetq, x_initial=[0 0 0 0]}
      mask prompts: b "Filter time constant"; x_initial "Initial output"
      mask help: Models a lag of the form 1/(b*s+1) where s is the Laplace operator.
  PID Controller : slpidlib/PID Controller  Controller=PID  Form=Parallel  TimeDomain=Continuous-time  UseExternalTs=off  SampleTime=-1  IntegratorMethod=Forward Euler  FilterMethod=Forward Euler  ControllerParametersSource=external  P=1  I=0  UseKiTs=off  D=0  UseExternalDerivativeSource=off  N=10  UseFilter=on  TunerSelectOption=Transfer Function Based (PID Tuner App)  InitialConditionSource=internal  InitialConditionForIntegrator=0  InitialConditionForFilter=0  DifferentiatorICPrevScaledInput=0  ExternalReset=none  TrackingMode=off  Kt=1  LimitOutput=on  SatLimitsSource=internal  UpperSaturationLimit=trq_max_pos  LowerSaturationLimit=trq_max_neg  LinearizeAsGain=on  AntiWindupMode=none  Kb=1  LimitIntegrator=off  UpperIntegratorSaturationLimit=inf  LowerIntegratorSaturationLimit=-inf  POutMin=[]  POutMax=[]  IOutMin=[]  IOutMax=[]  DOutMin=[]  DOutMax=[]  NOutMin=[]  NOutMax=[]  SumOutMin=[]  SumOutMax=[]  SaturationOutMin=[]  SaturationOutMax=[]  PParamMin=[]  PParamMax=[]  IParamMin=[]  IParamMax=[]  DParamMin=[]  DParamMax=[]  NParamMin=[]  NParamMax=[]  KbParamMin=[]  KbParamMax=[]  KtParamMin=[]  KtParamMax=[]  KbOutMin=[]  KbOutMax=[]  KtOutMin=[]  KtOutMax=[]  IntegratorOutMin=[]  IntegratorOutMax=[]  FilterOutMin=[]  FilterOutMax=[]  SumI1OutMin=[]  SumI1OutMax=[]  SumI2OutMin=[]  SumI2OutMax=[]  SumI3OutMin=[]  SumI3OutMax=[]  SumI4OutMin=[]  SumI4OutMax=[]  SumDOutMin=[]  SumDOutMax=[]  DifferentiatorOutMin=[]  DifferentiatorOutMax=[]  FilterDiffOutCoefMin=[]  FilterDiffOutCoefMax=[]  ReciprocalOutMin=[]  ReciprocalOutMax=[]  SumDenOutMin=[]  SumDenOutMax=[]  SumNumOutMin=[]  SumNumOutMax=[]  DivideOutMin=[]  DivideOutMax=[]  UdiffTsProdOutMin=[]  UdiffTsProdOutMax=[]  NTsProdOutMin=[]  NTsProdOutMax=[]  UintegralTsProdOutMin=[]  UintegralTsProdOutMax=[]  UngainTsProdOutMin=[]  UngainTsProdOutMax=[]  ClampingZeroOutDataTypeStr=Inherit: Inherit via back propagation  ClampingZeroOutMin=[]  ClampingZeroOutMax=[]  FilterDenConstantOutDataTypeStr=Inherit: Inherit via back propagation  FilterDenConstantOutMin=[]  FilterDenConstantOutMax=[]  PCopyOutDataTypeStr=Inherit: Inherit via back propagation  PCopyOutMin=[]  PCopyOutMax=[]  NCopyOutDataTypeStr=Inherit: Inherit via back propagation  NCopyOutMin=[]  NCopyOutMax=[]  IntegratorContinuousStateAttributes=''  IntegratorStateMustResolveToSignalObject=off  IntegratorRTWStateStorageClass=Auto  FilterContinuousStateAttributes=''  FilterStateMustResolveToSignalObject=off  FilterRTWStateStorageClass=Auto  ParallelPVariant=ExternalParameters  IdealPVariant=Disabled  IVariant=ExternalParameters  DVariant=ExternalParameters  IntegratorVariant=Continuous  SatVariant=Enabled  AWVariant=Passthrough  PCopyVariant=Disabled  TRVariant=Disabled  FdbkBlocksVariant=Forward  IdealPFdbkVariant=Disabled  SatFdbkVariant=Disabled  DerivativeFilterVariant=ContFilter  NVariant=ExternalParameters  NCopyVariant=Disabled  FilterICVariant=InternalICsFilter  IntegratorICVariant=InternalICs  ExternalResetVariant=Disabled  TRSumVariant=Passthrough  SumFdbkVariant=Disabled  SumVariant=Sum_PID  TsampFilterVariant=InternalTs  TsampNgainVariant=Passthrough  TsampIntegralVariant=Disabled_SignalSpec  ExternalSaturationOutDataTypeStr=Inherit: Same as second input  DerivativeSourceVariant=ErrorSignal  PreIntVariant=InternalPreInt
  Scope : Scope  NumInputPorts=4
      settings: ActiveDisplayYMinimum=-152.13979  ActiveDisplayYMaximum=38.47588
  Scope1 : Scope  NumInputPorts=4
      settings: ActiveDisplayYMinimum=-2.45349  ActiveDisplayYMaximum=1.54302  DataLoggingVariableName=ScopeData5
  Switch : Switch  Criteria=u2 > Threshold  SaturateOnIntegerOverflow=off  InputSameDT=off
  trq : Outport
  wires:
  PID Controller/1 -> trq/1
  qSteerWhl/1 -> Filter qTarget/1(In)
  Add/1 -> PID Controller/1, Demux1/1
  RoverAtGoal/1 -> Switch/2
  Constant1/1 -> Switch/1
  Demux/1 -> PID Controller/2
  Demux/2 -> PID Controller/3
  Constant/1 -> Switch/3
  Switch/1 -> Demux/1
  Meas/1 -> Bus to Vec/1(B)
  Bus to Vec/1(V) -> Filter qMeas/1(In)
  Check Difference/1(L3) -> Scope/1
  Check Difference/2(L1) -> Scope/2
  Check Difference/3(R3) -> Scope/3
  Check Difference/4(R1) -> Scope/4
  Constant2/1 -> PID Controller/4
  Filter qMeas/1(Out) -> Check Difference/2(meas), Add/2
  Filter qTarget/1(Out) -> Add/1, Check Difference/1(tgt)
  Demux1/1 -> Scope1/1
  Demux1/2 -> Scope1/2
  Demux1/3 -> Scope1/3
  Demux1/4 -> Scope1/4
  Constant3/1 -> PID Controller/5

== system mars_rover_terrain/Control/Chassis Control/Target Dir To Bicycle Steer Angle ==
  TargetDir : Inport
  Bicycle length : Constant  Value=L
  Constant : Constant  Value=2
  Divide : Product  Inputs=*/
  Lookahead distance : Constant  Value=ld
  Product : Product
  Product1 : Product
  Rad2Deg : MATLAB Function  TreatAsAtomicUnit=on
  Scope : Scope  NumInputPorts=4
      settings: ActiveDisplayYMinimum=-0.21556  ActiveDisplayYMaximum=0.02395  DataLoggingVariableName=ScopeData2
  Sine Wave : Sin  TimeSource=Use external signal  SampleTime=0
  Trigonometric Function : Trigonometry  Operator=atan
  qSteer : Outport
  wires:
  Sine Wave/1 -> Product1/2, Scope/2
  Bicycle length/1 -> Product/2
  Constant/1 -> Product/1
  Product1/1 -> Divide/1
  Product/1 -> Product1/1
  Divide/1 -> Trigonometric Function/1
  Trigonometric Function/1 -> Scope/3, Rad2Deg/1(u)
  TargetDir/1 -> Scope/1, Sine Wave/1
  Lookahead distance/1 -> Divide/2
  Rad2Deg/1(y) -> Scope/4, qSteer/1

== system mars_rover_terrain/Control/Chassis Control/Target Direction and Speed ==
  vRover : Inport
  Pose : Inport  Port=2
  WP : Inport  Port=3
  AND : Logic  IconShape=distinctive  AllPortsSameDT=off  OutDataTypeStr=boolean
  Check Distance To Goal : Subsystem
  Check for Stop : simulink/Logic and Bit Operations/Compare To Constant  relop=<=  const=0.05  OutDataTypeStr=boolean
  Clock3 : Clock
  Constant10 : Constant  Value=Control.Drive.StartTime
  Constant11 : Constant  Value=Control.Drive.TargetAccel
  Constant7 : Constant  Value=[rover_path.x(end) rover_path.y(end)]
  Demux : Demux  Outputs=3
  Pure Pursuit Control : robotalgslib/Pure Pursuit  DesiredLinearVelocityPort=off  DesiredLinearVelocity=Control.Drive.TargetSpeed  MaxAngularVelocity=0.01  LookaheadDistancePort=off  LookaheadDistance=0.75  TargetDirPort=on  SimulateUsing=Code generation
  Scope : Scope  NumInputPorts=2
      settings: ActiveDisplayYMinimum=-0.21027  ActiveDisplayYMaximum=0.31469  DataLoggingVariableName=ScopeData3
  Scope1 : Scope  NumInputPorts=3
      settings: ActiveDisplayYMinimum=56.41006  ActiveDisplayYMaximum=71.60549  DataLoggingVariableName=ScopeData4
  Terminator : Terminator
  Transfer Fcn : TransferFcn  Denominator=[0.1 1]
  Transfer Fcn1 : TransferFcn  Denominator=[0.5 1]
  Trapezoidal Vel Profile : MATLAB Function  TreatAsAtomicUnit=on
  hold : Subsystem
  StopAtGoal : Outport
  vTarget : Outport  Port=2
  AtGoal : Outport  Port=3
  TargetDir : Outport  Port=4
  wires:
  hold/1(Out1) -> Trapezoidal Vel Profile/4(deaccelStartTime)
  Pure Pursuit Control/1 -> Trapezoidal Vel Profile/5(linVel), Check Distance To Goal/3(linVel)
  Constant11/1 -> Trapezoidal Vel Profile/3(accel)
  Constant7/1 -> Check Distance To Goal/1(goal)
  Check Distance To Goal/1(atGoal) -> AtGoal/1, AND/2
  Clock3/1 -> Trapezoidal Vel Profile/1(t)
  Check for Stop/1 -> AND/1
  Pose/1 -> Demux/1, Check Distance To Goal/2(currentPose), Pure Pursuit Control/1
  Pure Pursuit Control/2 -> Terminator/1
  Constant10/1 -> Trapezoidal Vel Profile/2(startTime)
  Check Distance To Goal/2(Slow) -> hold/1(In1)
  AND/1 -> StopAtGoal/1
  WP/1 -> Pure Pursuit Control/2
  Trapezoidal Vel Profile/1(lin_Vel_out) -> Transfer Fcn/1
  Transfer Fcn/1 -> vTarget/1
  Transfer Fcn1/1 -> Scope/2, TargetDir/1
  vRover/1 -> Check for Stop/1
  Demux/1 -> Scope1/1
  Demux/2 -> Scope1/2
  Demux/3 -> Scope1/3
  Pure Pursuit Control/3 -> Scope/1, Transfer Fcn1/1

== system mars_rover_terrain/Control/Chassis Control/Vec to Bus SteerTrq ==
  V : Inport
  Bus Creator : BusCreator  Inputs=4
  Demux : Demux
  B : Outport
  wires:
  Demux/3 -> Bus Creator/3  "R3"
  Bus Creator/1 -> B/1
  V/1 -> Demux/1
  Demux/4 -> Bus Creator/4  "R1"
  Demux/1 -> Bus Creator/1  "L3"
  Demux/2 -> Bus Creator/2  "L1"

== system mars_rover_terrain/Control/Chassis Control/Vec to Bus qSteer ==
  V : Inport
  Bus Creator : BusCreator  Inputs=4
  Demux : Demux
  B : Outport
  wires:
  Demux/2 -> Bus Creator/2  "L1"
  Demux/4 -> Bus Creator/4  "R1"
  Demux/3 -> Bus Creator/3  "R3"
  Demux/1 -> Bus Creator/1  "L3"
  Bus Creator/1 -> B/1
  V/1 -> Demux/1

== system mars_rover_terrain/Control/Chassis Control/Vec to Bus trq ==
  V : Inport
  Bus Creator : BusCreator  Inputs=6
  Demux : Demux  Outputs=6
  B : Outport
  wires:
  Demux/5 -> Bus Creator/5  "R2"
  Demux/2 -> Bus Creator/2  "L2"
  Demux/6 -> Bus Creator/6  "R3"
  Demux/1 -> Bus Creator/1  "L1"
  Demux/4 -> Bus Creator/4  "R1"
  V/1 -> Demux/1
  Bus Creator/1 -> B/1
  Demux/3 -> Bus Creator/3  "L3"

== system mars_rover_terrain/Control/Chassis Control/Vec to Bus wWhl ==
  V : Inport
  Bus Creator : BusCreator  Inputs=6
  Demux : Demux  Outputs=6
  B : Outport
  wires:
  V/1 -> Demux/1
  Bus Creator/1 -> B/1
  Demux/1 -> Bus Creator/1  "L1"
  Demux/3 -> Bus Creator/3  "L3"
  Demux/4 -> Bus Creator/4  "R1"
  Demux/2 -> Bus Creator/2  "L2"
  Demux/5 -> Bus Creator/5  "R2"
  Demux/6 -> Bus Creator/6  "R3"

== system mars_rover_terrain/Control/Chassis Control/Wheel Speed Controller ==
  Meas : Inport
  StopAtGoal : Inport  Port=2
  wTarget : Inport  Port=3
  Add3 : Sum  Inputs=+-
  Bus to Vec : Subsystem
  Constant : Constant  Value=[Kp,Ki]
  Constant1 : Constant  Value=[5000 100]
  Constant2 : Constant  Value=Kd
  Constant3 : Constant  Value=N
  Demux : Demux  Outputs=2
  Filter wMeas : Subsystem  mask(First-order lag supporting vector signals){b=[1 1 1 1 1 1]*Ts_Measw, x_initial=[0 0 0 0 0 0]}
      mask prompts: b "Filter time constant"; x_initial "Initial output"
      mask help: Models a lag of the form 1/(b*s+1) where s is the Laplace operator.
  Filter wTarget : Subsystem  mask(First-order lag supporting vector signals){b=[1 1 1 1 1 1]*Ts_Targetw, x_initial=[0 0 0 0 0 0]}
      mask prompts: b "Filter time constant"; x_initial "Initial output"
      mask help: Models a lag of the form 1/(b*s+1) where s is the Laplace operator.
  PID Controller : slpidlib/PID Controller  Controller=PID  Form=Parallel  TimeDomain=Continuous-time  UseExternalTs=off  SampleTime=-1  IntegratorMethod=Forward Euler  FilterMethod=Forward Euler  ControllerParametersSource=external  P=1  I=0  UseKiTs=off  D=0  UseExternalDerivativeSource=off  N=100  UseFilter=on  TunerSelectOption=Transfer Function Based (PID Tuner App)  InitialConditionSource=internal  InitialConditionForIntegrator=0  InitialConditionForFilter=0  DifferentiatorICPrevScaledInput=0  ExternalReset=none  TrackingMode=off  Kt=1  LimitOutput=off  SatLimitsSource=internal  UpperSaturationLimit=inf  LowerSaturationLimit=-inf  LinearizeAsGain=on  AntiWindupMode=none  Kb=1  LimitIntegrator=off  UpperIntegratorSaturationLimit=inf  LowerIntegratorSaturationLimit=-inf  POutMin=[]  POutMax=[]  IOutMin=[]  IOutMax=[]  DOutMin=[]  DOutMax=[]  NOutMin=[]  NOutMax=[]  SumOutMin=[]  SumOutMax=[]  SaturationOutMin=[]  SaturationOutMax=[]  PParamMin=[]  PParamMax=[]  IParamMin=[]  IParamMax=[]  DParamMin=[]  DParamMax=[]  NParamMin=[]  NParamMax=[]  KbParamMin=[]  KbParamMax=[]  KtParamMin=[]  KtParamMax=[]  KbOutMin=[]  KbOutMax=[]  KtOutMin=[]  KtOutMax=[]  IntegratorOutMin=[]  IntegratorOutMax=[]  FilterOutMin=[]  FilterOutMax=[]  SumI1OutMin=[]  SumI1OutMax=[]  SumI2OutMin=[]  SumI2OutMax=[]  SumI3OutMin=[]  SumI3OutMax=[]  SumI4OutMin=[]  SumI4OutMax=[]  SumDOutMin=[]  SumDOutMax=[]  DifferentiatorOutMin=[]  DifferentiatorOutMax=[]  FilterDiffOutCoefMin=[]  FilterDiffOutCoefMax=[]  ReciprocalOutMin=[]  ReciprocalOutMax=[]  SumDenOutMin=[]  SumDenOutMax=[]  SumNumOutMin=[]  SumNumOutMax=[]  DivideOutMin=[]  DivideOutMax=[]  UdiffTsProdOutMin=[]  UdiffTsProdOutMax=[]  NTsProdOutMin=[]  NTsProdOutMax=[]  UintegralTsProdOutMin=[]  UintegralTsProdOutMax=[]  UngainTsProdOutMin=[]  UngainTsProdOutMax=[]  ClampingZeroOutDataTypeStr=Inherit: Inherit via back propagation  ClampingZeroOutMin=[]  ClampingZeroOutMax=[]  FilterDenConstantOutDataTypeStr=Inherit: Inherit via back propagation  FilterDenConstantOutMin=[]  FilterDenConstantOutMax=[]  PCopyOutDataTypeStr=Inherit: Inherit via back propagation  PCopyOutMin=[]  PCopyOutMax=[]  NCopyOutDataTypeStr=Inherit: Inherit via back propagation  NCopyOutMin=[]  NCopyOutMax=[]  IntegratorContinuousStateAttributes=''  IntegratorStateMustResolveToSignalObject=off  IntegratorRTWStateStorageClass=Auto  FilterContinuousStateAttributes=''  FilterStateMustResolveToSignalObject=off  FilterRTWStateStorageClass=Auto  ParallelPVariant=ExternalParameters  IdealPVariant=Disabled  IVariant=ExternalParameters  DVariant=ExternalParameters  IntegratorVariant=Continuous  SatVariant=Disabled  AWVariant=Passthrough  PCopyVariant=Disabled  TRVariant=Disabled  FdbkBlocksVariant=Forward  IdealPFdbkVariant=Disabled  SatFdbkVariant=Disabled  DerivativeFilterVariant=ContFilter  NVariant=ExternalParameters  NCopyVariant=Disabled  FilterICVariant=InternalICsFilter  IntegratorICVariant=InternalICs  ExternalResetVariant=Disabled  TRSumVariant=Passthrough  SumFdbkVariant=Disabled  SumVariant=Sum_PID  TsampFilterVariant=InternalTs  TsampNgainVariant=Passthrough  TsampIntegralVariant=Disabled_SignalSpec  ExternalSaturationOutDataTypeStr=Inherit: Same as second input  DerivativeSourceVariant=ErrorSignal  PreIntVariant=InternalPreInt
  Saturation : Saturate  UpperLimit=trq_max_pos  LowerLimit=trq_max_neg
  Switch : Switch  Criteria=u2 > Threshold  SaturateOnIntegerOverflow=off  InputSameDT=off
  trq : Outport
  wires:
  Switch/1 -> Demux/1
  Constant/1 -> Switch/3
  Constant1/1 -> Switch/1
  Demux/2 -> PID Controller/3
  Demux/1 -> PID Controller/2
  StopAtGoal/1 -> Switch/2
  PID Controller/1 -> Saturation/1
  Meas/1 -> Bus to Vec/1(B)
  Add3/1 -> PID Controller/1
  Saturation/1 -> trq/1
  Bus to Vec/1(V) -> Filter wMeas/1(In)
  wTarget/1 -> Filter wTarget/1(In)
  Constant2/1 -> PID Controller/4
  Constant3/1 -> PID Controller/5
  Filter wMeas/1(Out) -> Add3/2
  Filter wTarget/1(Out) -> Add3/1
